simulink model "test3"  (R2025b)
settings: Solver=VariableStepAuto  StartTime=0.0  StopTime=10.0  RelTol=1e-3
settings Model: Creator=Shriram  LastModifiedBy=Shriram

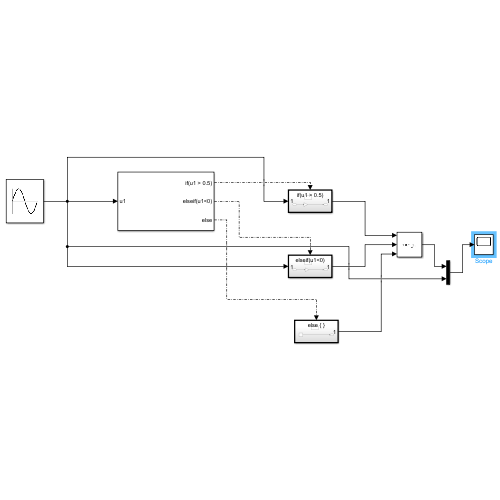
[thumbnail: Simulink's stored preview of the top-level diagram]
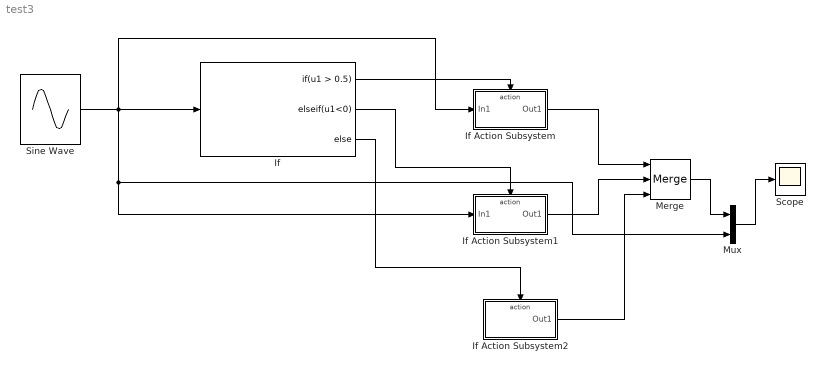
== system test3 ==
  If : If  IfExpression=u1 > 0.5  ElseIfExpressions=u1<0
  If Action Subsystem : Subsystem  TreatAsAtomicUnit=on
  If Action Subsystem1 : Subsystem  TreatAsAtomicUnit=on
  If Action Subsystem2 : Subsystem  TreatAsAtomicUnit=on
  Merge : Merge  Inputs=3
  Mux : Mux  Inputs=2
  Scope : Scope
      settings: ActiveDisplayYMinimum=-5.74808121368677  ActiveDisplayYMaximum=11.749786801520752
  Sine Wave : Sin  SampleTime=0
  wires:
  Sine Wave/1 -> Mux/2, If Action Subsystem1/1(In1), If Action Subsystem/1(In1), If/1
  If/1 -> If Action Subsystem/Action
  If/2 -> If Action Subsystem1/Action
  If/3 -> If Action Subsystem2/Action
  If Action Subsystem/1(Out1) -> Merge/1
  If Action Subsystem1/1(Out1) -> Merge/2
  If Action Subsystem2/1(Out1) -> Merge/3
  Merge/1 -> Mux/1
  Mux/1 -> Scope/1

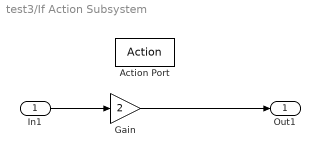
== system test3/If Action Subsystem ==
  In1 : Inport
  Action Port : ActionPort  ActionPortLabel=if(u1 > 0.5)
  Gain : Gain  Gain=2
  Out1 : Outport
  wires:
  In1/1 -> Gain/1
  Gain/1 -> Out1/1

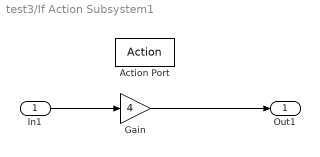
== system test3/If Action Subsystem1 ==
  In1 : Inport
  Action Port : ActionPort  ActionPortLabel=elseif(u1<0)
  Gain : Gain  Gain=4
  Out1 : Outport
  wires:
  In1/1 -> Gain/1
  Gain/1 -> Out1/1

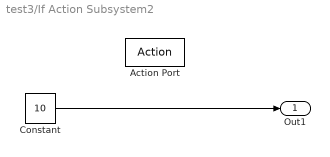
== system test3/If Action Subsystem2 ==
  Action Port : ActionPort  ActionPortLabel=else
  Constant : Constant  Value=10
  Out1 : Outport
  wires:
  Constant/1 -> Out1/1
